simulink model "vehicle_following"  (R2025b)
settings: Solver=VariableStepAuto  StartTime=0.0  StopTime=200.0  FixedStep=0.001  RelTol=1e-3
model workspace (MAT data in the model file):
  Kd = Simulink.Parameter
  Kd.Value = 0.01
  Kd.Complexity = 'real'
  Kd.Dimensions = [1 1]
  Kd.DataType = 'auto'
  Kp = Simulink.Parameter
  Kp.Value = 0.2
  Kp.Complexity = 'real'
  Kp.Dimensions = [1 1]
  Kp.DataType = 'auto'
  Ldes = Simulink.Parameter
  Ldes.Value = -30
  Ldes.Complexity = 'real'
  Ldes.Dimensions = [1 1]
  Ldes.DataType = 'auto'
  Ldes.DocUnits = 'ft'
settings Model: Creator=grantdahl  LastModifiedBy=grantdahl

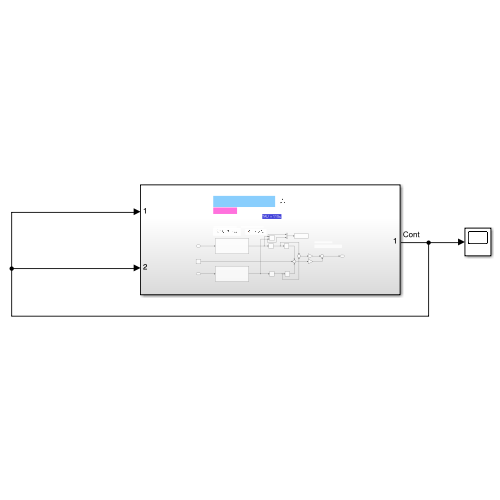
[thumbnail: Simulink's stored preview of the top-level diagram]
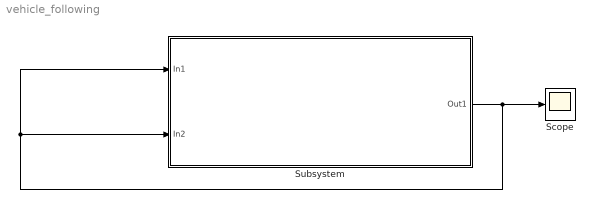
== system vehicle_following ==
  Scope : Scope
      settings: ActiveDisplayYMinimum=36.019999999998547  ActiveDisplayYMaximum=136.02000000001311
  Subsystem : Subsystem
  wires:
  Subsystem/1(Out1) -> Subsystem/2(In2), Subsystem/1(In1), Scope/1

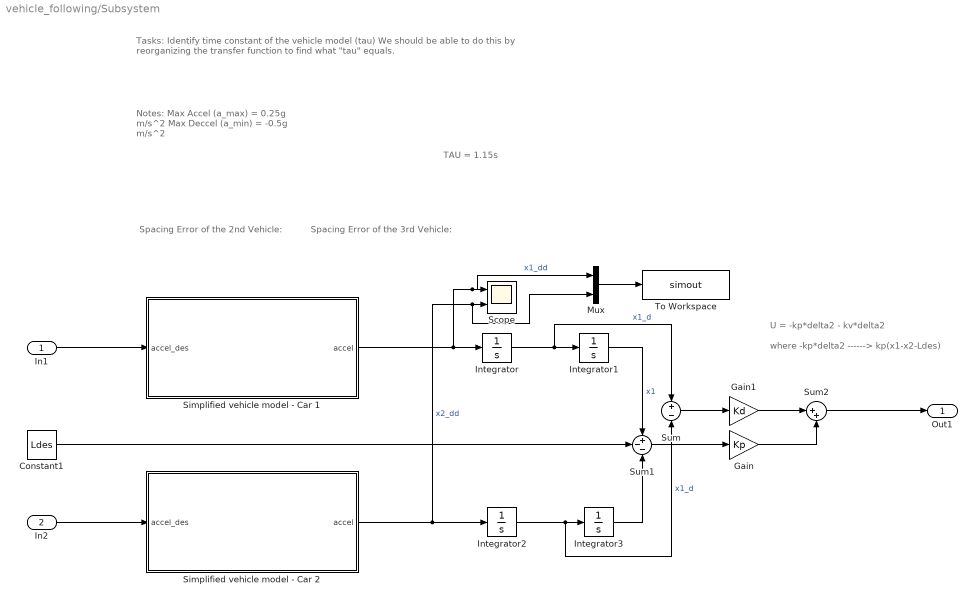
== system vehicle_following/Subsystem ==
  note: TAU = 1.15s
  note: where -kp*delta2 ------> kp(x1-x2-Ldes)
  note: U = -kp*delta2 - kv*delta2
  note: Spacing Error of the 2nd Vehicle:
  note: Notes:
      |
      | Max Accel (a_max) = 0.25g m/s^2
      | Max Deccel (a_min) = -0.5g m/s^2
  note: Tasks:
      |
      | Identify time constant of the vehicle model (tau)
      | 	We should be able to do this by reorganizing the transfer function to find what "tau" 		equals.
  note: Spacing Error of the 3rd Vehicle:
  In1 : Inport
  In2 : Inport  Port=2
  Constant1 : Constant  Value=Ldes
  Gain : Gain  Gain=Kp
  Gain1 : Gain  Gain=Kd
  Integrator : Integrator  InitialCondition=30
  Integrator1 : Integrator  InitialCondition=400
  Integrator2 : Integrator  InitialCondition=28
  Integrator3 : Integrator  InitialCondition=200
  Mux : Mux  Inputs=2
  Scope : Scope  NumInputPorts=2
      settings: ActiveDisplayYMinimum=-0.12499999999999997  ActiveDisplayYMaximum=1.125
  Simplified vehicle model - Car 1 : Subsystem  mask(Vehicle model){}
      mask help: Vehicle model
      mask Display: image('sedan.png');
  Simplified vehicle model - Car 2 : Subsystem  mask(Vehicle model){}
      mask help: Vehicle model
      mask Display: image('convertible.png');
  Sum : Sum  Inputs=+|-
  Sum1 : Sum  Inputs=+--
  Sum2 : Sum  Inputs=|++
  To Workspace : ToWorkspace  VariableName=simout  SaveFormat=Timeseries  SampleTime=-1
  Out1 : Outport
  wires:
  In2/1 -> Simplified vehicle model - Car 2/1(accel_des)
  Integrator3/1 -> Sum1/3
  In1/1 -> Simplified vehicle model - Car 1/1(accel_des)
  Constant1/1 -> Sum1/2
  Integrator/1 -> Sum/1, Integrator1/1  "x1_d"
  Sum1/1 -> Gain/1
  Integrator1/1 -> Sum1/1  "x1"
  Simplified vehicle model - Car 2/1(accel) -> Integrator2/1, Mux/2, Scope/2  "x2_dd"
  Integrator2/1 -> Sum/2, Integrator3/1  "x1_d"
  Simplified vehicle model - Car 1/1(accel) -> Mux/1, Scope/1, Integrator/1  "x1_dd"
  Sum/1 -> Gain1/1
  Gain1/1 -> Sum2/1
  Gain/1 -> Sum2/2
  Sum2/1 -> Out1/1
  Mux/1 -> To Workspace/1

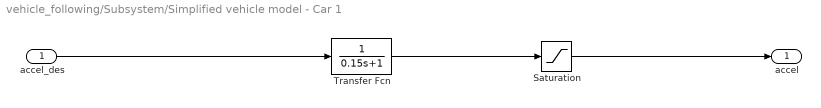
== system vehicle_following/Subsystem/Simplified vehicle model - Car 1 ==
  accel_des : Inport
  Saturation : Saturate  UpperLimit=2.5  LowerLimit=-5
  Transfer Fcn : TransferFcn  Denominator=[0.15 1]
  accel : Outport
  wires:
  Saturation/1 -> accel/1
  Transfer Fcn/1 -> Saturation/1
  accel_des/1 -> Transfer Fcn/1

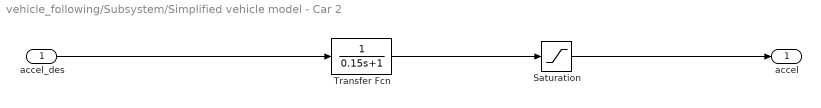
== system vehicle_following/Subsystem/Simplified vehicle model - Car 2 ==
  accel_des : Inport
  Saturation : Saturate  UpperLimit=2.5  LowerLimit=-5
  Transfer Fcn : TransferFcn  Denominator=[0.15 1]
  accel : Outport
  wires:
  Saturation/1 -> accel/1
  Transfer Fcn/1 -> Saturation/1
  accel_des/1 -> Transfer Fcn/1
